simulink model "Obstacle_avoidance_bot"  (R2024b)
settings: Solver=VariableStepAuto  StartTime=0.0  StopTime=30  MaxStep=0.01  RelTol=1e-3
libraries: simulink x1
settings Model: SimulationMode=accelerator  Creator=Grishma  LastModifiedBy=Grishma

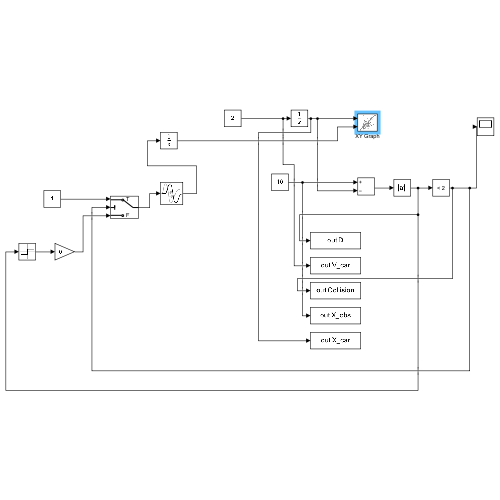
[thumbnail: Simulink's stored preview of the top-level diagram]
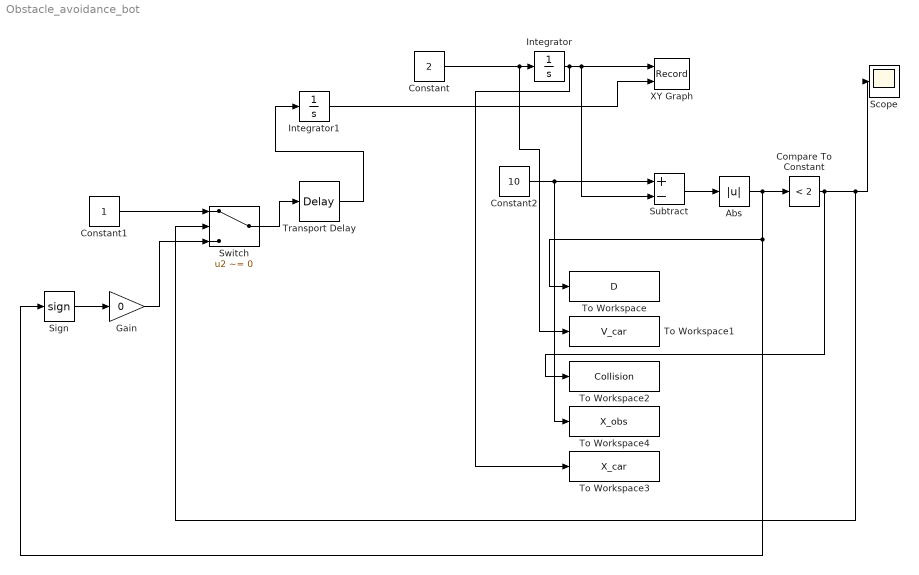
== system Obstacle_avoidance_bot ==
  Abs : Abs  SaturateOnIntegerOverflow=off
  Compare To Constant : simulink/Logic and Bit Operations/Compare To Constant  relop=<  const=2  OutDataTypeStr=boolean
  Constant : Constant  Value=2
  Constant1 : Constant
  Constant2 : Constant  Value=10
  Gain : Gain  Gain=0
  Integrator : Integrator
  Integrator1 : Integrator
  Scope : Scope
  Sign : Signum
  Subtract : Sum  Inputs=+-
  Switch : Switch  Criteria=u2 ~= 0  Threshold=0.5  SaturateOnIntegerOverflow=off  InputSameDT=off
  To Workspace : ToWorkspace  VariableName=D  SaveFormat=Structure With Time  SampleTime=-1
  To Workspace1 : ToWorkspace  VariableName=V_car  SaveFormat=Structure With Time  SampleTime=-1
  To Workspace2 : ToWorkspace  VariableName=Collision  SaveFormat=Structure With Time  SampleTime=-1
  To Workspace3 : ToWorkspace  VariableName=X_car  SaveFormat=Structure With Time  SampleTime=-1
  To Workspace4 : ToWorkspace  VariableName=X_obs  SaveFormat=Structure With Time  SampleTime=-1
  Transport Delay : TransportDelay
  XY Graph : Record  FileSettingsInternal="{\"entries\":[{\"content\":{\"excelSettings\":{\"content\":{},\"type\":\"Streamout.ExcelSettings\"}},\"type\":\"Streamout.FileSettingStorage\",\"uuid\":\"\"}],\"packageUris\":[\"http:\\/\\/schema.mathworks.com\\/mf0\\/streamout_blocks\\/R2020a\"],\"version\":\"1.0\"}"  Layout=[1 1]  SignalsInternal="{\"entries\":[{\"content\":{\"signals\":[{\"content\":{\"blockPath\":[],\"dimensions\":[1],\"domain\":\"\",\"lineColor\":\"#a2142f\",\"plots\":[ 1 ],\"port\":1,\"sid\":[\"\"],\"signalID\":1,\"signalName\":\"Integrator\"},\"type\":\"RecordBlkView.Signal\",\"uuid\":\"\"},{\"content\":{\"blockPath\":[],\"dimensions\":[1],\"domain\":\"\",\"lineColor\":\"#139fff\",\"plots\":[ 1 ],\"port\":2,\"sid\":[\"\"],\"signalID\":2,\"signalName\":\"Integrator1\"},\"type\":\"RecordBlkView.Signal\",\"uuid\":\"\"}]},\"type\":\"RecordBlkView.InputSignals\",\"uuid\":\"\"}],\"packageUris\":[\"http:\\/\\/schema.mathworks.com\\/mf0\\/streamout_blocks\\/R2020a\"],\"version\":\"1.0\"}"  VisualizationBindings="{\"xyplotplugin\":{\"info\":[{\"series\":[{\"bindingParametersList\":[{\"parameter\":\"X-Axis\",\"signalID\":1,\"signalName\":\"Integrator\"},{\"parameter\":\"Y-Axis\",\"signalID\":2,\"signalName\":\"Integrator1\"}],\"seriesID\":0}],\"subplotID\":1}]}}"  CompatibilityTag=XY
  wires:
  Constant/1 -> To Workspace1/1, Integrator/1
  Integrator/1 -> To Workspace3/1, Subtract/2, XY Graph/1
  Constant2/1 -> To Workspace4/1, Subtract/1
  Subtract/1 -> Abs/1
  Abs/1 -> Sign/1, To Workspace/1, Compare To Constant/1
  Compare To Constant/1 -> To Workspace2/1, Switch/2, Scope/1
  Integrator1/1 -> XY Graph/2
  Constant1/1 -> Switch/1
  Sign/1 -> Gain/1
  Gain/1 -> Switch/3
  Switch/1 -> Transport Delay/1
  Transport Delay/1 -> Integrator1/1
